simulink model "buck_plant"  (R2026b)
settings: Solver=FixedStepDiscrete  StopTime=0.1  FixedStep=TsPlant
values from neighbouring files (symbols this model uses):
  Ad = Mz(1:3, 1:3)    [buck_plant_params.m]    (also in check_buck_plant.m = expm(A*Ts))
  Bd = Mz(1:3, 4:5)    [buck_plant_params.m]    (also in check_buck_plant.m = A\((Ad - eye(2))*B))
  Cd = eye(3)    [buck_plant_params.m]
  Dd = zeros(3, 2)    [buck_plant_params.m]
  iL0 = 0    [buck_plant_params.m]
  TsPlant = 1/(58e3/2/3)    (= 0.000103448275862)    [buck_plant_params.m]
  vC0 = 0    [buck_plant_params.m]
settings Model: Creator=BenjaminRupp  LastModifiedBy=BenjaminRupp

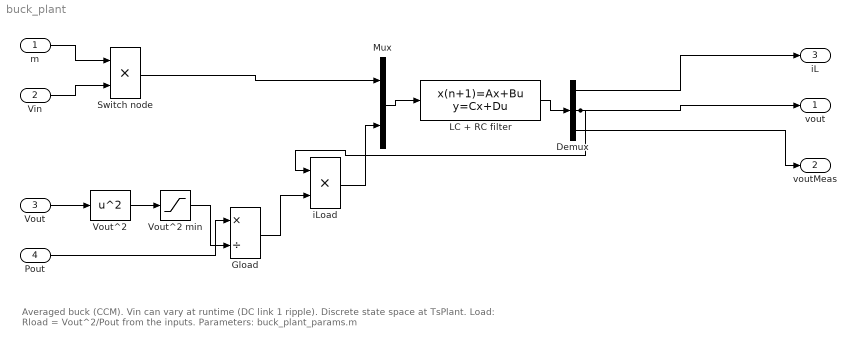
== system buck_plant ==
  note: Averaged buck (CCM). Vin can vary at runtime (DC link 1 ripple).
      | Discrete state space at TsPlant. Load: Rload = Vout^2/Pout from the inputs. Parameters: buck_plant_params.m
  m : Inport  Interpolate=off
  Vin : Inport  Port=2  Interpolate=off
  Vout : Inport  Port=3  Interpolate=off
  Pout : Inport  Port=4  Interpolate=off
  Demux : Demux  Outputs=3
  Gload : Product  Description=Load conductance 1/Rload = Pout/Vout^2  Inputs=*/
  LC + RC filter : DiscreteStateSpace  Description=x = [iL; vC; vMeas], u = [m*Vin; iLoad], exact ZOH at TsPlant (buck_plant_params.m)  A=Ad  B=Bd  C=Cd  D=Dd  InitialCondition=[iL0; vC0; vC0]  SampleTime=TsPlant
  Mux : Mux  Inputs=2
  Switch node : Product  Description=Averaged switch-node voltage m*Vin  Inputs=**
  Vout^2 : Math  Operator=square
  Vout^2 min : Saturate  UpperLimit=inf  LowerLimit=1
  iLoad : Product  Inputs=**
  vout : Outport
  voutMeas : Outport  Port=2
  iL : Outport  Port=3
  wires:
  m/1 -> Switch node/1
  Vin/1 -> Switch node/2
  Switch node/1 -> Mux/1
  Vout/1 -> Vout^2/1
  Vout^2/1 -> Vout^2 min/1
  Pout/1 -> Gload/1
  Vout^2 min/1 -> Gload/2
  Gload/1 -> iLoad/2
  Demux/2 -> iLoad/1, vout/1
  iLoad/1 -> Mux/2
  Mux/1 -> LC + RC filter/1
  LC + RC filter/1 -> Demux/1
  Demux/1 -> iL/1
  Demux/3 -> voutMeas/1
